simulink model "experiment_supervisor"  (R2025b)
settings: Solver=FixedStepDiscrete  StartTime=0.0  StopTime=inf  FixedStep=Ts  RelTol=1e-3
model workspace (MAT data in the model file):
  Ts = Simulink.Parameter
  Ts.Value = 0.01
  Ts.Complexity = 'real'
  Ts.Dimensions = [1 1]
  Ts.DataType = 'auto'
  Ts.DocUnits = 's'
  board_ID = Simulink.Parameter
  board_ID.Value = 1
  board_ID.Complexity = 'real'
  board_ID.Dimensions = [1 1]
  board_ID.DataType = 'auto'
undefined symbols (not defined in the file or in its folder): CAN_ANGLE_DEG2ICUB, CAN_ANGLE_ICUB2DEG, canChannel
libraries: canmsglib x21, canlib x4, simulink x1
settings Model: DataDictionary=amcbldc.sldd  Creator=upattacini  LastModifiedBy=rpumpo
settings SolverCC: AlgebraicLoopSolver=TrustRegion  DecoupledContinuousIntegration=on  MinimalZcImpactIntegration=on
settings OptimizationCC: ReuseModelBlockBuffer=off  SimCompilerOptimization=on
settings DebuggingCC: ParameterPrecisionLossMsg=none  UnconnectedInputMsg=warning  UnconnectedOutputMsg=warning  UnconnectedLineMsg=warning  ArithmeticOperatorsInVariantConditions=warning
settings HardwareCC: ProdBitPerLong=64.0  ProdHWDeviceType=Intel->x86-64 (Linux 64)
settings ModelReferenceCC: EnableRefExpFcnMdlSchedulingChecks=on
settings SFSimCC: SimUseLocalCustomCode=off  CustomCodeUndefinedFunction=UseInterfaceOnly
settings RTWCC: SystemTargetFile=sldrt.tlc  TemplateMakefile=sldrt.tmf  RTWUseLocalCustomCode=off  RTWCompilerOptimization=on  GPUComputeCapability=3.5  DLArmComputeVersion=19.05  Description=Simulink Desktop Real-Time
settings CodeAppCC: MaxIdLength=95.0
settings SimulinkDesktopRealTimeCC: ExtModeTransport=0.0  ExtModeStaticAllocSize=1000000.0  TargetLibSuffix=_sldrt.a  TargetPreCompLibLocation=C:\Program Files\MATLAB\R2025b\toolbox\sldrt\lib\win64  MultiwordLength=2048.0  DynamicStringBufferSize=256.0  ParMdlRefBuildCompliant=on  PreserveMATLABNamespacesInGeneratedCode=on  SubcomponentCodeInterfacePackaging=Reusable function

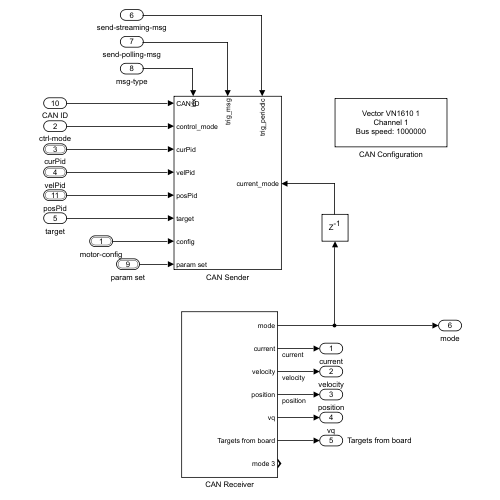
[thumbnail: Simulink's stored preview of the top-level diagram]
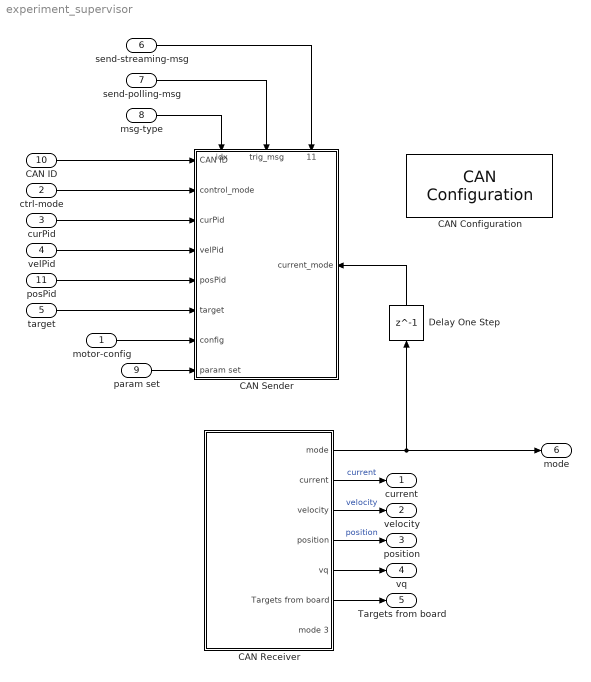
== system experiment_supervisor ==
  motor-config : Inport  OutDataTypeStr=Bus: MotorConfigurationExternal
  ctrl-mode : Inport  Port=2  OutDataTypeStr=Enum: MCControlModes
  curPid : Inport  Port=3  OutDataTypeStr=Bus: PID
  velPid : Inport  Port=4  OutDataTypeStr=Bus: PID
  target : Inport  Port=5
  send-streaming-msg : Inport  Port=6  OutDataTypeStr=uint8
  send-polling-msg : Inport  Port=7  OutDataTypeStr=uint8
  msg-type : Inport  Port=8  OutDataTypeStr=uint8
  param set : Inport  Port=9  OutDataTypeStr=Bus: MotorConfigurationExtSet
  CAN ID : Inport  Port=10
  posPid : Inport  Port=11  OutDataTypeStr=Bus: PID
  CAN Configuration : canlib/CAN Configuration  BlockHandle=6361.001  Device=Vector VN1610 1 (Channel 1)  DeviceMenu=Vector VN1610 1 (Channel 1)  ObjConstructor=canChannel('Vector', 'VN1610 1', 1)  BusSpeed=1000000  EnableBitParameters=off  SJW=1  TSEG1=4  TSEG2=3  NSamples=1  AckMode=Normal
  CAN Receiver : Subsystem
  CAN Sender : Subsystem
      settings: PortSchema="{\"entries\":[{\"content\":{\"sides\":[{\"content\":{\"connectorIds\":[\"In1\",\"In2\",\"In3\",\"In4\",\"In5\",\"In6\",\"In7\",\"In8\"]},\"type\":\"ConnectorPlacement.EquallySpacedRectSide\",\"uuid\":\"bdd6ce9e-9b65-4aba-9b48-f09f8c1326bb\"},{\"content\":{\"connectorIds\":[\"In12\"],\"side\":\"RIGHT\"},\"type\":\"ConnectorPlacement.EquallySpacedRectSide\",\"uuid\":\"141c9ef5-f742-47fc-b635-015c7474b58f\"},{\"content\":{\"connectorIds\":[\"In9\",\"In10\",\"In11\"],\"side\":\"TOP\"},\"type\":\"ConnectorPlacement.EquallySpacedRectSide\",\"uuid\":\"624889ac-74c5-4b05-9d21-0587daea952f\"}]},\"type\":\"ConnectorPlacement.EquallySpacedConnector\",\"uuid\":\"a748afda-e52d-41b4-a312-ee668058905d\"}],\"packageUris\":[\"http://schema.mathworks.com/mf0/Connector/R2020b\"],\"version\":\"1.0\"}"
  Delay One Step : Delay  DelayLength=1
  current : Outport
  velocity : Outport  Port=2
  position : Outport  Port=3
  vq : Outport  Port=4
  Targets from board : Outport  Port=5
  mode : Outport  Port=6
  wires:
  CAN Receiver/2(current) -> current/1  "current"
  CAN Receiver/3(velocity) -> velocity/1  "velocity"
  CAN Receiver/4(position) -> position/1  "position"
  CAN Receiver/5(vq) -> vq/1
  ctrl-mode/1 -> CAN Sender/2(control_mode)
  send-streaming-msg/1 -> CAN Sender/11(trig_periodic)
  CAN Receiver/6(Targets from board) -> Targets from board/1
  velPid/1 -> CAN Sender/4(velPid)
  curPid/1 -> CAN Sender/3(curPid)
  motor-config/1 -> CAN Sender/7(config)
  Delay One Step/1 -> CAN Sender/12(current_mode)
  send-polling-msg/1 -> CAN Sender/10(trig_msg)
  msg-type/1 -> CAN Sender/9(idx)
  target/1 -> CAN Sender/6(target)
  CAN ID/1 -> CAN Sender/1(CAN ID)
  CAN Receiver/1(mode) -> Delay One Step/1, mode/1
  param set/1 -> CAN Sender/8(param set)
  posPid/1 -> CAN Sender/5(posPid)

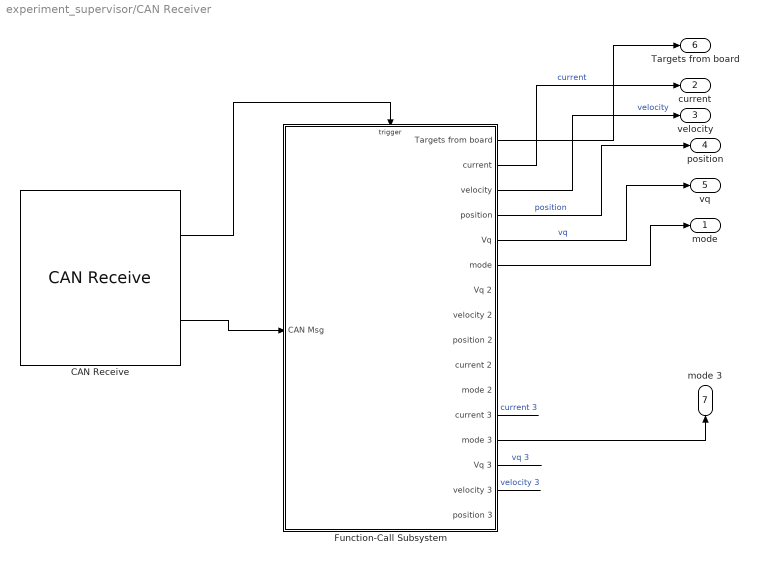
== system experiment_supervisor/CAN Receiver ==
  CAN Receive : canlib/CAN Receive  BlockHandle=6370.0007  Device=Vector VN1610 1 (Channel 1)  DeviceMenu=Vector VN1610 1 (Channel 1)  ObjConstructor=canChannel('Vector', 'VN1610 1', 1)  EnableStandardIDsFilter=off  StdIDsCombo=Allow all  StandardIDs=0  EnableExtendedIDsFilter=off  ExtIDsCombo=Allow all  ExtendedIDs=0  SampleTime=Ts  MsgsPerTimestep=all  InternalFilterUpdateStatus=on  BusOutput=on
  Function-Call Subsystem : Subsystem  TreatAsAtomicUnit=on
  mode : Outport
  current : Outport  Port=2
  velocity : Outport  Port=3
  position : Outport  Port=4
  vq : Outport  Port=5
  Targets from board : Outport  Port=6
  mode 3 : Outport  Port=7
  wires:
  CAN Receive/1 -> Function-Call Subsystem/Trigger
  CAN Receive/2 -> Function-Call Subsystem/1(CAN Msg)
  Function-Call Subsystem/2(current) -> current/1  "current"
  Function-Call Subsystem/3(velocity) -> velocity/1  "velocity"
  Function-Call Subsystem/4(position) -> position/1  "position"
  Function-Call Subsystem/5(Vq) -> vq/1  "vq"
  Function-Call Subsystem/1(Targets from board) -> Targets from board/1
  Function-Call Subsystem/6(mode) -> mode/1
  Function-Call Subsystem/12(current 3) -> ?  "current 3"
  Function-Call Subsystem/14(Vq 3) -> ?  "vq 3"
  Function-Call Subsystem/15(velocity 3) -> ?  "velocity 3"
  Function-Call Subsystem/13(mode 3) -> mode 3/1

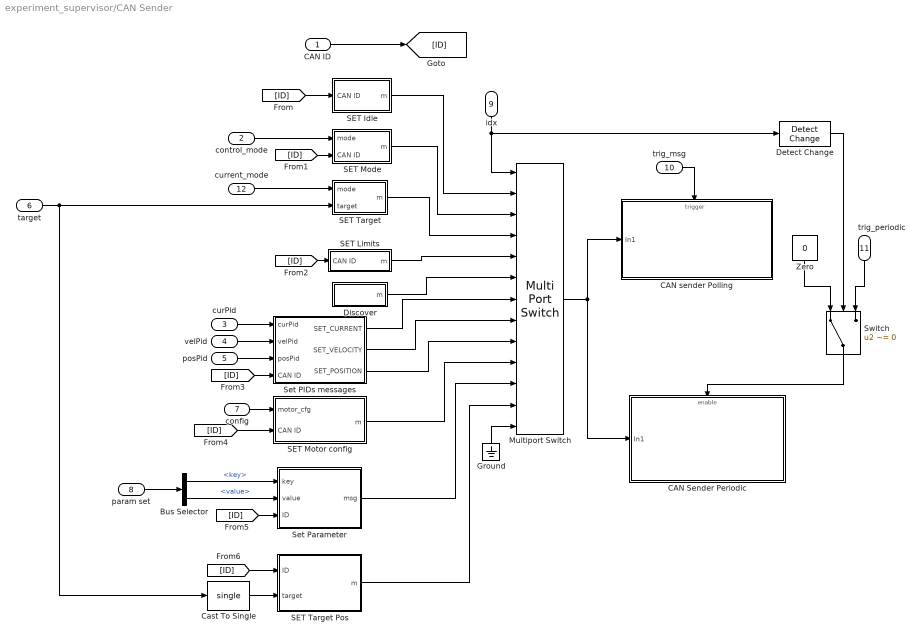
== system experiment_supervisor/CAN Sender ==
  CAN ID : Inport
  control_mode : Inport  Port=2
  curPid : Inport  Port=3
  velPid : Inport  Port=4
  posPid : Inport  Port=5
  target : Inport  Port=6
  config : Inport  Port=7
  param set : Inport  Port=8  OutDataTypeStr=Bus: MotorConfigurationExtSet
  idx : Inport  Port=9
  trig_msg : Inport  Port=10
  trig_periodic : Inport  Port=11
  current_mode : Inport  Port=12
  Bus Selector : BusSelector  OutputSignals=key,value
  CAN Sender Periodic : Subsystem  TreatAsAtomicUnit=on
  CAN sender Polling : Subsystem
  Cast To Single : DataTypeConversion  OutDataTypeStr=single  SaturateOnIntegerOverflow=off  RndMeth=Floor
  Detect Change : simulink/Logic and Bit Operations/Detect Change  vinit=0  OutDataTypeStr=boolean
  Discover : Subsystem
  Ground : Ground
  Multiport Switch : MultiPortSwitch  Inputs=11  DataPortForDefault=Additional data port  DiagnosticForDefault=None  SaturateOnIntegerOverflow=off  InputSameDT=off
  SET Idle : Subsystem
  SET Limits : Subsystem
  SET Mode : Subsystem
  SET Motor config : Subsystem
  SET Target : Subsystem
  SET Target Pos : Subsystem
  Set PIDs messages : Subsystem
  Set Parameter : Subsystem
  Switch : Switch  Criteria=u2 ~= 0  SaturateOnIntegerOverflow=off  InputSameDT=off
  Zero : Constant  Value=0  OutDataTypeStr=Inherit: Inherit via back propagation
  wires:
  idx/1 -> Multiport Switch/1, Detect Change/1
  trig_msg/1 -> CAN sender Polling/Trigger
  trig_periodic/1 -> Switch/3
  Multiport Switch/1 -> CAN sender Polling/1(In1), CAN Sender Periodic/1(In1)
  Set PIDs messages/2(SET_VELOCITY) -> Multiport Switch/8
  Set PIDs messages/1(SET_CURRENT) -> Multiport Switch/7
  velPid/1 -> Set PIDs messages/2(velPid)
  curPid/1 -> Set PIDs messages/1(curPid)
  Detect Change/1 -> Switch/2
  Zero/1 -> Switch/1
  Switch/1 -> CAN Sender Periodic/Enable
  SET Limits/1(m) -> Multiport Switch/5
  current_mode/1 -> SET Target/1(mode)
  target/1 -> Cast To Single/1, SET Target/2(target)
  SET Target/1(m) -> Multiport Switch/4
  config/1 -> SET Motor config/1(motor_cfg)
  SET Motor config/1(m) -> Multiport Switch/10
  control_mode/1 -> SET Mode/1(mode)
  SET Mode/1(m) -> Multiport Switch/3
  SET Idle/1(m) -> Multiport Switch/2
  Discover/1(m) -> Multiport Switch/6
  [ID] -> SET Idle/1(CAN ID)
  [ID] -> SET Mode/2(CAN ID)
  [ID] -> SET Limits/1(CAN ID)
  [ID] -> Set PIDs messages/4(CAN ID)
  [ID] -> SET Motor config/2(CAN ID)
  CAN ID/1 -> [ID]
  Set Parameter/1(msg) -> Multiport Switch/11
  [ID] -> Set Parameter/3(ID)
  param set/1 -> Bus Selector/1
  Bus Selector/1 -> Set Parameter/1(key)  "<key>"
  Bus Selector/2 -> Set Parameter/2(value)  "<value>"
  posPid/1 -> Set PIDs messages/3(posPid)
  Ground/1 -> Multiport Switch/13
  Set PIDs messages/3(SET_POSITION) -> Multiport Switch/9
  Cast To Single/1 -> SET Target Pos/2(target)
  [ID] -> SET Target Pos/1(ID)
  SET Target Pos/1(m) -> Multiport Switch/12

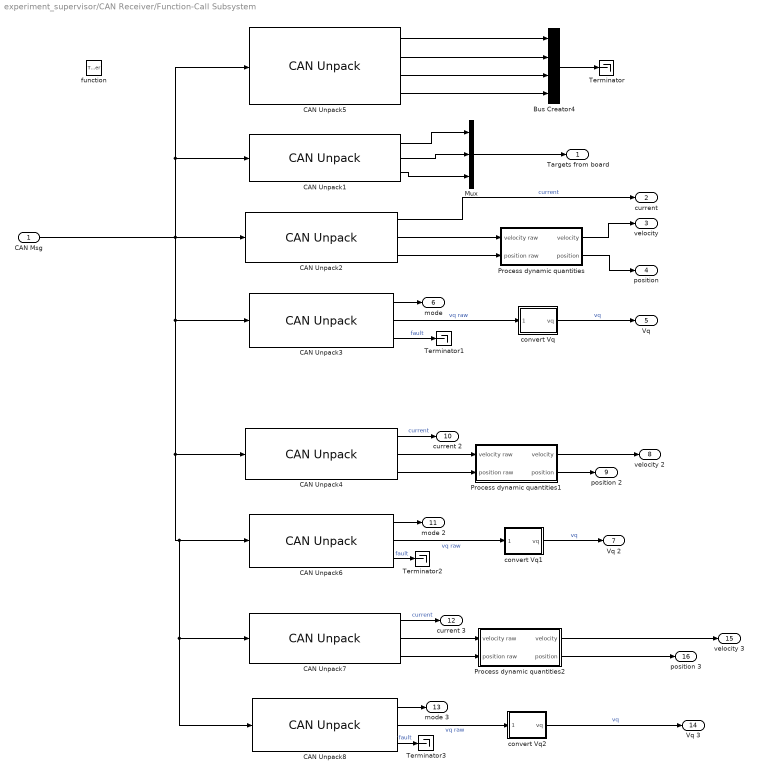
== system experiment_supervisor/CAN Receiver/Function-Call Subsystem ==
  CAN Msg : Inport
  function : TriggerPort  TriggerType=function-call  VariantControl=(inherit)
  Bus Creator4 : BusCreator  Inputs=4
  CAN Unpack1 : canmsglib/CAN Unpack  MsgList=(none)  MsgName=TARGETS  MsgIDType=Standard (11-bit identifier)  MsgIdentifier=0x10F  MsgLength=8  SignalInfo={ 'Target1', '0', '16', 'LE', 'signed', 'Standard', '0', '1', '0', '-Inf', 'Inf'; 'Target2', '16', '16', 'LE', 'signed', 'Standard', '0', '1', '0', '-Inf', 'Inf'; 'Target3', '32', '16', 'LE', 'signed', 'Standard', '0', '1', '0', '-Inf', 'Inf' }  IDPort=off  TimestampPort=off  ErrorPort=off  RemotePort=off  LengthPort=off  StatusPort=off  ApplyMinMax=off
  CAN Unpack2 : canmsglib/CAN Unpack  MsgList=(none)  MsgName=FOC  MsgIDType=Standard (11-bit identifier)  MsgIdentifier=0x110  MsgLength=8  SignalInfo={ 'current', '0', '16', 'LE', 'signed', 'Standard', '0', '1', '0', '-Inf', 'Inf'; 'velocity', '16', '16', 'LE', 'signed', 'Standard', '0', '1', '0', '-Inf', 'Inf'; 'position', '32', '32', 'LE', 'signed', 'Standard', '0', '1', '0', '-Inf', 'Inf' }  IDPort=off  TimestampPort=off  ErrorPort=off  RemotePort=off  LengthPort=off  StatusPort=off  ApplyMinMax=off
  CAN Unpack3 : canmsglib/CAN Unpack  MsgList=(none)  MsgName=STATUS  MsgIDType=Standard (11-bit identifier)  MsgIdentifier=0x113  MsgLength=8  SignalInfo={ 'mode', '0', '8', 'LE', 'unsigned', 'Standard', '0', '1', '0', '-Inf', 'Inf'; 'pwm', '16', '16', 'LE', 'unsigned', 'Standard', '0', '1', '0', '-Inf', 'Inf'; 'fault', '32', '8', 'LE', 'unsigned', 'Standard', '0', '1', '0', '-Inf', 'Inf' }  IDPort=off  TimestampPort=off  ErrorPort=off  RemotePort=off  LengthPort=off  StatusPort=off  ApplyMinMax=off
  CAN Unpack4 : canmsglib/CAN Unpack  MsgList=(none)  MsgName=FOC  MsgIDType=Standard (11-bit identifier)  MsgIdentifier=0x120  MsgLength=8  SignalInfo={ 'current', '0', '16', 'LE', 'signed', 'Standard', '0', '1', '0', '-Inf', 'Inf'; 'velocity', '16', '16', 'LE', 'signed', 'Standard', '0', '1', '0', '-Inf', 'Inf'; 'position', '32', '32', 'LE', 'signed', 'Standard', '0', '1', '0', '-Inf', 'Inf' }  IDPort=off  TimestampPort=off  ErrorPort=off  RemotePort=off  LengthPort=off  StatusPort=off  ApplyMinMax=off
  CAN Unpack5 : canmsglib/CAN Unpack  MsgList=(none)  MsgName=DISCOVER  MsgIDType=Standard (11-bit identifier)  MsgIdentifier=0x710  MsgLength=5  SignalInfo={}  IDPort=on  TimestampPort=on  ErrorPort=off  RemotePort=off  LengthPort=on  StatusPort=off  ApplyMinMax=off
      settings: DataFormat=raw data
  CAN Unpack6 : canmsglib/CAN Unpack  MsgList=(none)  MsgName=STATUS  MsgIDType=Standard (11-bit identifier)  MsgIdentifier=0x123  MsgLength=8  SignalInfo={ 'mode', '0', '8', 'LE', 'unsigned', 'Standard', '0', '1', '0', '-Inf', 'Inf'; 'pwm', '16', '16', 'LE', 'unsigned', 'Standard', '0', '1', '0', '-Inf', 'Inf'; 'fault', '32', '8', 'LE', 'unsigned', 'Standard', '0', '1', '0', '-Inf', 'Inf' }  IDPort=off  TimestampPort=off  ErrorPort=off  RemotePort=off  LengthPort=off  StatusPort=off  ApplyMinMax=off
  CAN Unpack7 : canmsglib/CAN Unpack  MsgList=(none)  MsgName=FOC  MsgIDType=Standard (11-bit identifier)  MsgIdentifier=0x130  MsgLength=8  SignalInfo={ 'current', '0', '16', 'LE', 'signed', 'Standard', '0', '1', '0', '-Inf', 'Inf'; 'velocity', '16', '16', 'LE', 'signed', 'Standard', '0', '1', '0', '-Inf', 'Inf'; 'position', '32', '32', 'LE', 'signed', 'Standard', '0', '1', '0', '-Inf', 'Inf' }  IDPort=off  TimestampPort=off  ErrorPort=off  RemotePort=off  LengthPort=off  StatusPort=off  ApplyMinMax=off
  CAN Unpack8 : canmsglib/CAN Unpack  MsgList=(none)  MsgName=STATUS  MsgIDType=Standard (11-bit identifier)  MsgIdentifier=0x133  MsgLength=8  SignalInfo={ 'mode', '0', '8', 'LE', 'unsigned', 'Standard', '0', '1', '0', '-Inf', 'Inf'; 'pwm', '16', '16', 'LE', 'unsigned', 'Standard', '0', '1', '0', '-Inf', 'Inf'; 'fault', '32', '8', 'LE', 'unsigned', 'Standard', '0', '1', '0', '-Inf', 'Inf' }  IDPort=off  TimestampPort=off  ErrorPort=off  RemotePort=off  LengthPort=off  StatusPort=off  ApplyMinMax=off
  Mux : Mux  Inputs=3
  Process dynamic quantities : Subsystem
  Process dynamic quantities1 : Subsystem
  Process dynamic quantities2 : Subsystem
  Terminator{,1..3} (4 alike) : Terminator
  convert Vq : Subsystem
  convert Vq1 : Subsystem
  convert Vq2 : Subsystem
  Targets from board : Outport
  current : Outport  Port=2  Unit=mA
  velocity : Outport  Port=3  Unit=deg/s
  position : Outport  Port=4  Unit=deg
  Vq : Outport  Port=5  Unit=%  PortDimensions=1
  mode : Outport  Port=6  OutDataTypeStr=uint8
  Vq 2 : Outport  Port=7
  velocity 2 : Outport  Port=8
  position 2 : Outport  Port=9
  current 2 : Outport  Port=10  Unit=mA
  mode 2 : Outport  Port=11  OutDataTypeStr=uint8
  current 3 : Outport  Port=12  Unit=mA
  mode 3 : Outport  Port=13  OutDataTypeStr=uint8
  Vq 3 : Outport  Port=14
  velocity 3 : Outport  Port=15
  position 3 : Outport  Port=16
  wires:
  CAN Unpack5/4 -> Bus Creator4/4
  CAN Unpack5/3 -> Bus Creator4/3
  CAN Unpack5/2 -> Bus Creator4/2
  CAN Unpack5/1 -> Bus Creator4/1
  Bus Creator4/1 -> Terminator/1
  CAN Unpack1/1 -> Mux/1
  CAN Unpack1/2 -> Mux/2
  CAN Unpack1/3 -> Mux/3
  Mux/1 -> Targets from board/1
  CAN Unpack2/2 -> Process dynamic quantities/1(velocity raw)
  CAN Unpack2/1 -> current/1  "current"
  Process dynamic quantities/2(position) -> position/1
  Process dynamic quantities/1(velocity) -> velocity/1
  CAN Unpack2/3 -> Process dynamic quantities/2(position raw)
  CAN Unpack3/2 -> convert Vq/1(vq raw)  "vq raw"
  CAN Unpack3/1 -> mode/1
  convert Vq/1(vq) -> Vq/1  "vq"
  CAN Unpack3/3 -> Terminator1/1  "fault"
  CAN Unpack4/2 -> Process dynamic quantities1/1(velocity raw)
  CAN Unpack4/3 -> Process dynamic quantities1/2(position raw)
  CAN Unpack6/2 -> convert Vq1/1(vq raw)  "vq raw"
  Process dynamic quantities1/1(velocity) -> velocity 2/1
  Process dynamic quantities1/2(position) -> position 2/1
  convert Vq1/1(vq) -> Vq 2/1  "vq"
  CAN Unpack4/1 -> current 2/1  "current"
  CAN Unpack6/1 -> mode 2/1
  CAN Unpack6/3 -> Terminator2/1  "fault"
  CAN Unpack8/3 -> Terminator3/1  "fault"
  CAN Unpack8/2 -> convert Vq2/1(vq raw)  "vq raw"
  CAN Unpack7/3 -> Process dynamic quantities2/2(position raw)
  CAN Unpack7/1 -> current 3/1  "current"
  CAN Unpack8/1 -> mode 3/1
  CAN Unpack7/2 -> Process dynamic quantities2/1(velocity raw)
  CAN Msg/1 -> CAN Unpack5/1, CAN Unpack1/1, CAN Unpack8/1, CAN Unpack7/1, CAN Unpack6/1, CAN Unpack4/1, CAN Unpack3/1, CAN Unpack2/1
  Process dynamic quantities2/2(position) -> position 3/1
  Process dynamic quantities2/1(velocity) -> velocity 3/1
  convert Vq2/1(vq) -> Vq 3/1  "vq"

== system experiment_supervisor/CAN Sender/CAN Sender Periodic ==
  In1 : Inport
  Enable : EnablePort
  CAN Transmit : canlib/CAN Transmit  BlockHandle=6815.0006  Device=Vector VN1610 1 (Channel 1)  DeviceMenu=Vector VN1610 1 (Channel 1)  ObjConstructor=canChannel('Vector', 'VN1610 1', 1)  EnableEventTransmit=off  EnablePeriodicTransmit=on  MessagePeriod=Ts
  wires:
  In1/1 -> CAN Transmit/1

== system experiment_supervisor/CAN Sender/CAN sender Polling ==
  In1 : Inport
  Trigger : TriggerPort  VariantControl=(inherit)  PortDimensions=1
  CAN Transmit : canlib/CAN Transmit  BlockHandle=6832.001  Device=Vector VN1610 1 (Channel 1)  DeviceMenu=Vector VN1610 1 (Channel 1)  ObjConstructor=canChannel('Vector', 'VN1610 1', 1)  EnableEventTransmit=off  EnablePeriodicTransmit=off  MessagePeriod=1.000
  wires:
  In1/1 -> CAN Transmit/1

== system experiment_supervisor/CAN Sender/Discover ==
  CAN Pack4 : canmsglib/CAN Pack  MsgList=(none)  MsgName=DISCOVER  MsgIDType=Standard (11-bit identifier)  MsgIdentifier=0x70F  CANIDInput=off  MsgLength=1  Remote=off  ApplyMinMax=off  BusOutput=on  SignalInfo={}
      settings: DataFormat=raw data
  discover : Constant  Value=0xFF
  m : Outport
  wires:
  CAN Pack4/1 -> m/1
  discover/1 -> CAN Pack4/1

== system experiment_supervisor/CAN Sender/SET Idle ==
  CAN ID : Inport
  CAN Pack : canmsglib/CAN Pack  MsgList=(none)  MsgName=CAN Idle  MsgIDType=Standard (11-bit identifier)  MsgIdentifier=board_ID  CANIDInput=on  MsgLength=2  Remote=off  ApplyMinMax=off  BusOutput=on  SignalInfo={ 'Idle', '0', '16', 'LE', 'unsigned', 'Standard', '0', '1', '0', '-Inf', 'Inf' }
      settings: DataFormat=manually specified signals
  idle-mode : Constant  Value=0x09  OutDataTypeStr=Inherit: Inherit via back propagation
  m : Outport
  wires:
  idle-mode/1 -> CAN Pack/1
  CAN ID/1 -> CAN Pack/2
  CAN Pack/1 -> m/1

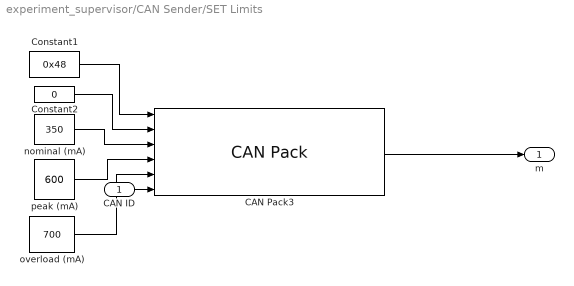
== system experiment_supervisor/CAN Sender/SET Limits ==
  CAN ID : Inport
  CAN Pack3 : canmsglib/CAN Pack  MsgList=(none)  MsgName=CAN Limits  MsgIDType=Standard (11-bit identifier)  MsgIdentifier=board_ID  CANIDInput=on  MsgLength=8  Remote=off  ApplyMinMax=off  BusOutput=on  SignalInfo={ 'CMD', '0', '8', 'LE', 'unsigned', 'Standard', '0', '1', '0', '-Inf', 'Inf'; 'X', '8', '8', 'LE', 'unsigned', 'Standard', '0', '1', '0', '-Inf', 'Inf'; 'NOMINAL', '16', '16', 'LE', 'unsigned', 'Standard', '0', '1', '0', '-Inf', 'Inf'; 'PEAK', '32', '16', 'LE', 'unsigned', 'Standard', '0', '1', '0', '-Inf', 'Inf'; 'OVERLOAD', '48', '16', 'LE', 'unsigned', 'Standard', '0', '1', '0', '-Inf', 'Inf' }
      settings: DataFormat=manually specified signals
  Constant1 : Constant  Value=0x48  OutDataTypeStr=Inherit: Inherit via back propagation
  Constant2 : Constant  Value=0  OutDataTypeStr=Inherit: Inherit via back propagation
  nominal (mA) : Constant  Value=350  OutDataTypeStr=Inherit: Inherit via back propagation
  overload (mA) : Constant  Value=700  OutDataTypeStr=Inherit: Inherit via back propagation
  peak (mA) : Constant  Value=600  OutDataTypeStr=Inherit: Inherit via back propagation
  m : Outport
  wires:
  Constant2/1 -> CAN Pack3/2
  Constant1/1 -> CAN Pack3/1
  nominal (mA)/1 -> CAN Pack3/3
  overload (mA)/1 -> CAN Pack3/5
  peak (mA)/1 -> CAN Pack3/4
  CAN ID/1 -> CAN Pack3/6
  CAN Pack3/1 -> m/1

== system experiment_supervisor/CAN Sender/SET Mode ==
  mode : Inport
  CAN ID : Inport  Port=2
  CAN Pack1 : canmsglib/CAN Pack  MsgList=(none)  MsgName=SET Control Mode  MsgIDType=Standard (11-bit identifier)  MsgIdentifier=board_ID  CANIDInput=on  MsgLength=2  Remote=off  ApplyMinMax=off  BusOutput=on  SignalInfo={ 'CMD', '0', '8', 'LE', 'unsigned', 'Standard', '0', '1', '0', '-Inf', 'Inf'; 'CTRL', '8', '8', 'LE', 'signed', 'Standard', '0', '1', '0', '-Inf', 'Inf' }
      settings: DataFormat=manually specified signals
  Cast : DataTypeConversion  OutDataTypeStr=uint8  SaturateOnIntegerOverflow=off  RndMeth=Floor
  current-mode : Constant  Value=0x09  OutDataTypeStr=Inherit: Inherit via back propagation
  m : Outport
  wires:
  current-mode/1 -> CAN Pack1/1
  Cast/1 -> CAN Pack1/2
  mode/1 -> Cast/1
  CAN ID/1 -> CAN Pack1/3
  CAN Pack1/1 -> m/1

== system experiment_supervisor/CAN Sender/SET Motor config ==
  motor_cfg : Inport
  CAN ID : Inport  Port=2
  CAN Pack5 : canmsglib/CAN Pack  MsgList=(none)  MsgName=Set_Motor_Config  MsgIDType=Standard (11-bit identifier)  MsgIdentifier=board_ID  CANIDInput=on  MsgLength=8  Remote=off  ApplyMinMax=off  BusOutput=on  SignalInfo={ 'CMD', '0', '8', 'LE', 'unsigned', 'Standard', '0', '1', '0', '-Inf', 'Inf'; 'FLAGS', '8', '8', 'LE', 'unsigned', 'Standard', '0', '1', '0', '-Inf', 'Inf'; 'RES_ENCODER', '16', '16', 'LE', 'signed', 'Standard', '0', '1', '0', '-Inf', 'Inf'; 'OFFSET_ENCODER', '32', '16', 'LE', 'unsigned', 'Standard', '0', '1', '0', '-Inf', 'Inf'; 'N_POLES', '48', '8', 'LE', 'unsigned', 'Standard', '0', '1', '0', '-Inf', 'Inf'; 'ENCODER_TOLERANCE', '56', '8', 'LE', 'unsigned', 'Standard', '0', '1', '0', '-Inf', 'Inf' }
      settings: DataFormat=manually specified signals
  Constant3 : Constant  Value=0x77  OutDataTypeStr=Inherit: Inherit via back propagation
  Unpack motor configuration : MATLAB Function  TreatAsAtomicUnit=on
  m : Outport
  wires:
  motor_cfg/1 -> Unpack motor configuration/1(motor_cfg)
  Unpack motor configuration/2(resolution) -> CAN Pack5/3
  Unpack motor configuration/3(rotor_offset) -> CAN Pack5/4
  Unpack motor configuration/1(flags) -> CAN Pack5/2
  Unpack motor configuration/4(n_poles) -> CAN Pack5/5
  Unpack motor configuration/5(enc_tolerance) -> CAN Pack5/6
  Constant3/1 -> CAN Pack5/1
  CAN ID/1 -> CAN Pack5/7
  CAN Pack5/1 -> m/1

== system experiment_supervisor/CAN Sender/SET Target ==
  mode : Inport
  target : Inport  Port=2
  CAN Pack2 : canmsglib/CAN Pack  MsgList=(none)  MsgName=CAN Target  MsgIDType=Standard (11-bit identifier)  MsgIdentifier=0x10F  CANIDInput=off  MsgLength=8  Remote=off  ApplyMinMax=off  BusOutput=on  SignalInfo={ 'Target 1', '0', '16', 'LE', 'signed', 'Standard', '0', '1', '0', '-Inf', 'Inf'; 'Target 2', '16', '16', 'LE', 'signed', 'Standard', '0', '1', '0', '-Inf', 'Inf'; 'Target 3', '32', '16', 'LE', 'signed', 'Standard', '0', '1', '0', '-Inf', 'Inf'; 'Target 4', '48', '16', 'LE', 'signed', 'Standard', '0', '1', '0', '-Inf', 'Inf' }
      settings: DataFormat=manually specified signals
  Cast To Single : DataTypeConversion  OutDataTypeStr=single  SaturateOnIntegerOverflow=off  RndMeth=Floor
  Cast1 : DataTypeConversion  OutDataTypeStr=Enum: MCControlModes  SaturateOnIntegerOverflow=off  RndMeth=Floor
  Target conditioning : Subsystem
  m : Outport
  wires:
  Target conditioning/1(out) -> CAN Pack2/1, CAN Pack2/2, CAN Pack2/4, CAN Pack2/3  "target"
  Cast To Single/1 -> Target conditioning/2(tg)
  Cast1/1 -> Target conditioning/1(control_mode)
  target/1 -> Cast To Single/1
  CAN Pack2/1 -> m/1
  mode/1 -> Cast1/1

== system experiment_supervisor/CAN Sender/SET Target Pos ==
  ID : Inport
  target : Inport  Port=2
  CAN Pack2 : canmsglib/CAN Pack  MsgList=(none)  MsgName=SET  MsgIDType=Standard (11-bit identifier)  MsgIdentifier=0x10F  CANIDInput=on  MsgLength=8  Remote=off  ApplyMinMax=off  BusOutput=on  SignalInfo={ 'CMD', '0', '8', 'LE', 'unsigned', 'Standard', '0', '1', '0', '-Inf', 'Inf'; 'SetPos', '8', '8', 'LE', 'unsigned', 'Standard', '0', '1', '0', '-Inf', 'Inf'; 'TargetPos', '16', '32', 'LE', 'single', 'Standard', '0', '1', '0', '-Inf', 'Inf'; 'Vel', '48', '16', 'LE', 'unsigned', 'Standard', '0', '1', '0', '-Inf', 'Inf' }
      settings: DataFormat=manually specified signals
  Constant : Constant  Value=0x70e2  OutDataTypeStr=uint16
  Constant1 : Constant  Value=0x05
  Target conditioning : Subsystem
  m : Outport
  wires:
  target/1 -> Target conditioning/1(tg)
  CAN Pack2/1 -> m/1
  ID/1 -> CAN Pack2/5
  Constant/1 -> CAN Pack2/4
  Constant1/1 -> CAN Pack2/1
  Target conditioning/1(ID) -> CAN Pack2/2
  Target conditioning/2(Position) -> CAN Pack2/3

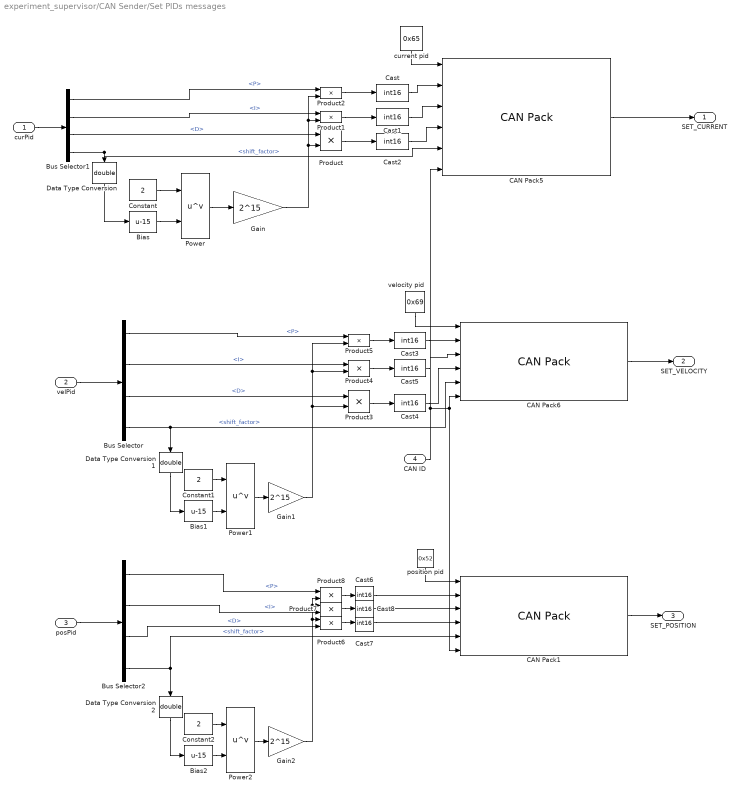
== system experiment_supervisor/CAN Sender/Set PIDs messages ==
  curPid : Inport
  velPid : Inport  Port=2
  posPid : Inport  Port=3
  CAN ID : Inport  Port=4
  Bias : Bias  Bias=-15  SaturateOnIntegerOverflow=off
  Bias1 : Bias  Bias=-15  SaturateOnIntegerOverflow=off
  Bias2 : Bias  Bias=-15  SaturateOnIntegerOverflow=off
  Bus Selector : BusSelector  OutputSignals=P,I,D,shift_factor
  Bus Selector1 : BusSelector  OutputSignals=P,I,D,shift_factor
  Bus Selector2 : BusSelector  OutputSignals=P,I,D,shift_factor
  CAN Pack1 : canmsglib/CAN Pack  MsgList=(none)  MsgName=SET_VELOCITY_PID  MsgIDType=Standard (11-bit identifier)  MsgIdentifier=board_ID  CANIDInput=on  MsgLength=8  Remote=off  ApplyMinMax=off  BusOutput=on  SignalInfo={ 'CMD', '0', '8', 'LE', 'unsigned', 'Standard', '0', '1', '0', '-Inf', 'Inf'; 'Kp', '8', '16', 'LE', 'signed', 'Standard', '0', '1', '0', '-Inf', 'Inf'; 'Ki', '24', '16', 'LE', 'signed', 'Standard', '0', '1', '0', '-Inf', 'Inf'; 'Kd', '40', '16', 'LE', 'signed', 'Standard', '0', '1', '0', '-Inf', 'Inf'; 'shift', '56', '8', 'LE', 'unsigned', 'Standard', '0', '1', '0', '-Inf', 'Inf' }
      settings: DataFormat=manually specified signals
  CAN Pack5 : canmsglib/CAN Pack  MsgList=(none)  MsgName=SET_CURRENT_PID  MsgIDType=Standard (11-bit identifier)  MsgIdentifier=board_ID  CANIDInput=on  MsgLength=8  Remote=off  ApplyMinMax=off  BusOutput=on  SignalInfo={ 'CMD', '0', '8', 'LE', 'unsigned', 'Standard', '0', '1', '0', '-Inf', 'Inf'; 'Kp', '8', '16', 'LE', 'signed', 'Standard', '0', '1', '0', '-Inf', 'Inf'; 'Ki', '24', '16', 'LE', 'signed', 'Standard', '0', '1', '0', '-Inf', 'Inf'; 'Kd', '40', '16', 'LE', 'signed', 'Standard', '0', '1', '0', '-Inf', 'Inf'; 'shift', '56', '8', 'LE', 'unsigned', 'Standard', '0', '1', '0', '-Inf', 'Inf' }
      settings: DataFormat=manually specified signals
  CAN Pack6 : canmsglib/CAN Pack  MsgList=(none)  MsgName=SET_VELOCITY_PID  MsgIDType=Standard (11-bit identifier)  MsgIdentifier=board_ID  CANIDInput=on  MsgLength=8  Remote=off  ApplyMinMax=off  BusOutput=on  SignalInfo={ 'CMD', '0', '8', 'LE', 'unsigned', 'Standard', '0', '1', '0', '-Inf', 'Inf'; 'Kp', '8', '16', 'LE', 'signed', 'Standard', '0', '1', '0', '-Inf', 'Inf'; 'Ki', '24', '16', 'LE', 'signed', 'Standard', '0', '1', '0', '-Inf', 'Inf'; 'Kd', '40', '16', 'LE', 'signed', 'Standard', '0', '1', '0', '-Inf', 'Inf'; 'shift', '56', '8', 'LE', 'unsigned', 'Standard', '0', '1', '0', '-Inf', 'Inf' }
      settings: DataFormat=manually specified signals
  Cast{,1..8} (9 alike) : DataTypeConversion  OutDataTypeStr=int16  SaturateOnIntegerOverflow=off  RndMeth=Floor
  Constant : Constant  Value=2
  Constant1 : Constant  Value=2
  Constant2 : Constant  Value=2
  Data Type Conversion : DataTypeConversion  OutDataTypeStr=double  SaturateOnIntegerOverflow=off  RndMeth=Floor
  Data Type Conversion1 : DataTypeConversion  OutDataTypeStr=double  SaturateOnIntegerOverflow=off  RndMeth=Floor
  Data Type Conversion2 : DataTypeConversion  OutDataTypeStr=double  SaturateOnIntegerOverflow=off  RndMeth=Floor
  Gain : Gain  Gain=2^15  OutDataTypeStr=single
  Gain1 : Gain  Gain=2^15  OutDataTypeStr=single
  Gain2 : Gain  Gain=2^15  OutDataTypeStr=single
  Power : Math  Operator=pow
  Power1 : Math  Operator=pow
  Power2 : Math  Operator=pow
  Product{,1..8} (9 alike) : Product
  current pid : Constant  Value=0x65  OutDataTypeStr=int16
  position pid : Constant  Value=0x52  OutDataTypeStr=int16
  velocity pid : Constant  Value=0x69  OutDataTypeStr=int16
  SET_CURRENT : Outport
  SET_VELOCITY : Outport  Port=2
  SET_POSITION : Outport  Port=3
  wires:
  Bus Selector/4 -> CAN Pack6/5, Data Type Conversion1/1  "<shift_factor>"
  Bus Selector1/4 -> CAN Pack5/5, Data Type Conversion/1  "<shift_factor>"
  Bus Selector1/1 -> Product2/1  "<P>"
  Bus Selector1/2 -> Product1/1  "<I>"
  current pid/1 -> CAN Pack5/1
  velocity pid/1 -> CAN Pack6/1
  CAN Pack5/1 -> SET_CURRENT/1
  CAN Pack6/1 -> SET_VELOCITY/1
  velPid/1 -> Bus Selector/1
  curPid/1 -> Bus Selector1/1
  Bus Selector1/3 -> Product/1  "<D>"
  Power/1 -> Gain/1
  Gain/1 -> Product2/2, Product1/2, Product/2
  Product/1 -> Cast2/1
  Product1/1 -> Cast1/1
  Product2/1 -> Cast/1
  Cast/1 -> CAN Pack5/2
  Cast1/1 -> CAN Pack5/3
  Cast2/1 -> CAN Pack5/4
  Constant/1 -> Power/1
  Bias/1 -> Power/2
  Data Type Conversion/1 -> Bias/1
  Cast5/1 -> CAN Pack6/3
  Bus Selector/2 -> Product4/1  "<I>"
  Cast3/1 -> CAN Pack6/2
  Bus Selector/3 -> Product3/1  "<D>"
  Bus Selector/1 -> Product5/1  "<P>"
  Cast4/1 -> CAN Pack6/4
  CAN ID/1 -> CAN Pack6/6, CAN Pack1/6, CAN Pack5/6
  position pid/1 -> CAN Pack1/1
  posPid/1 -> Bus Selector2/1
  Gain1/1 -> Product3/2, Product5/2, Product4/2
  Bias1/1 -> Power1/2
  Data Type Conversion1/1 -> Bias1/1
  Constant1/1 -> Power1/1
  Power1/1 -> Gain1/1
  Product5/1 -> Cast3/1
  Product4/1 -> Cast5/1
  Product3/1 -> Cast4/1
  Constant2/1 -> Power2/1
  Bias2/1 -> Power2/2
  Data Type Conversion2/1 -> Bias2/1
  Gain2/1 -> Product8/2, Product7/1, Product6/1
  Power2/1 -> Gain2/1
  Bus Selector2/4 -> Data Type Conversion2/1, CAN Pack1/5  "<shift_factor>"
  Product6/1 -> Cast7/1
  Product8/1 -> Cast6/1
  Product7/1 -> Cast8/1
  Cast6/1 -> CAN Pack1/2
  Cast8/1 -> CAN Pack1/3
  Cast7/1 -> CAN Pack1/4
  Bus Selector2/3 -> Product6/2  "<D>"
  Bus Selector2/2 -> Product7/2  "<I>"
  Bus Selector2/1 -> Product8/1  "<P>"
  CAN Pack1/1 -> SET_POSITION/1

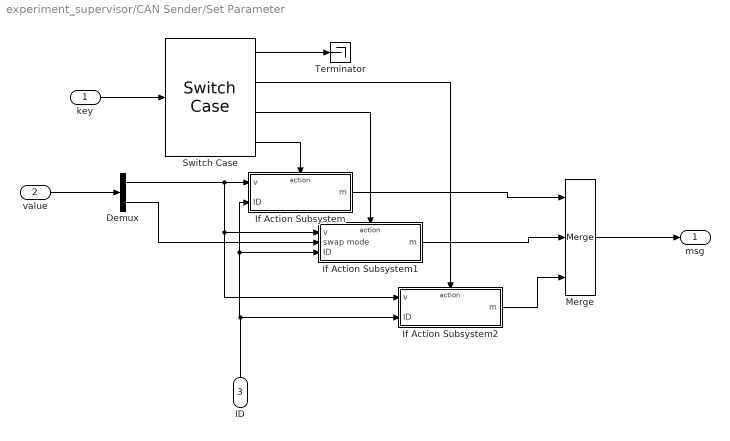
== system experiment_supervisor/CAN Sender/Set Parameter ==
  key : Inport
  value : Inport  Port=2
  ID : Inport  Port=3
  Demux : Demux  Outputs=2
  If Action Subsystem : Subsystem  TreatAsAtomicUnit=on
  If Action Subsystem1 : Subsystem  TreatAsAtomicUnit=on
  If Action Subsystem2 : Subsystem  TreatAsAtomicUnit=on
  Merge : Merge  Inputs=3
  Switch Case : SwitchCase  CaseConditions="{MCMotorParamsSet.None, MCMotorParamsSet.Kbemf, MCMotorParamsSet.hall,  MCMotorParamsSet.elect_vmax}"  ShowDefaultCase=off
  Terminator : Terminator
  msg : Outport
  wires:
  Merge/1 -> msg/1
  If Action Subsystem/1(m) -> Merge/1
  Demux/1 -> If Action Subsystem2/1(v), If Action Subsystem1/1(v), If Action Subsystem/1(v)
  key/1 -> Switch Case/1
  If Action Subsystem1/1(m) -> Merge/2
  If Action Subsystem2/1(m) -> Merge/3
  ID/1 -> If Action Subsystem/2(ID), If Action Subsystem1/3(ID), If Action Subsystem2/2(ID)
  Demux/2 -> If Action Subsystem1/2(swap mode)
  value/1 -> Demux/1
  Switch Case/2 -> If Action Subsystem2/Action
  Switch Case/3 -> If Action Subsystem1/Action
  Switch Case/4 -> If Action Subsystem/Action
  Switch Case/1 -> Terminator/1

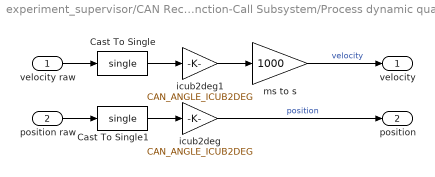
== system experiment_supervisor/CAN Receiver/Function-Call Subsystem/Process dynamic quantities ==
  velocity raw : Inport
  position raw : Inport  Port=2
  Cast To Single : DataTypeConversion  OutDataTypeStr=single  SaturateOnIntegerOverflow=off  RndMeth=Floor
  Cast To Single1 : DataTypeConversion  OutDataTypeStr=single  SaturateOnIntegerOverflow=off  RndMeth=Floor
  icub2deg : Gain  Gain=CAN_ANGLE_ICUB2DEG
  icub2deg1 : Gain  Gain=CAN_ANGLE_ICUB2DEG
  ms to s : Gain  Gain=1000
  velocity : Outport
  position : Outport  Port=2
  wires:
  Cast To Single1/1 -> icub2deg/1
  icub2deg1/1 -> ms to s/1
  Cast To Single/1 -> icub2deg1/1
  icub2deg/1 -> position/1  "position"
  velocity raw/1 -> Cast To Single/1
  position raw/1 -> Cast To Single1/1
  ms to s/1 -> velocity/1  "velocity"

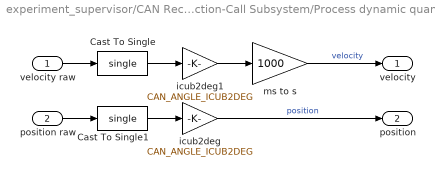
== system experiment_supervisor/CAN Receiver/Function-Call Subsystem/Process dynamic quantities1 ==
  velocity raw : Inport
  position raw : Inport  Port=2
  Cast To Single : DataTypeConversion  OutDataTypeStr=single  SaturateOnIntegerOverflow=off  RndMeth=Floor
  Cast To Single1 : DataTypeConversion  OutDataTypeStr=single  SaturateOnIntegerOverflow=off  RndMeth=Floor
  icub2deg : Gain  Gain=CAN_ANGLE_ICUB2DEG
  icub2deg1 : Gain  Gain=CAN_ANGLE_ICUB2DEG
  ms to s : Gain  Gain=1000
  velocity : Outport
  position : Outport  Port=2
  wires:
  Cast To Single1/1 -> icub2deg/1
  icub2deg1/1 -> ms to s/1
  Cast To Single/1 -> icub2deg1/1
  icub2deg/1 -> position/1  "position"
  velocity raw/1 -> Cast To Single/1
  position raw/1 -> Cast To Single1/1
  ms to s/1 -> velocity/1  "velocity"

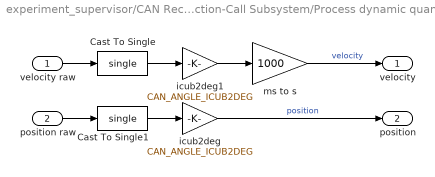
== system experiment_supervisor/CAN Receiver/Function-Call Subsystem/Process dynamic quantities2 ==
  velocity raw : Inport
  position raw : Inport  Port=2
  Cast To Single : DataTypeConversion  OutDataTypeStr=single  SaturateOnIntegerOverflow=off  RndMeth=Floor
  Cast To Single1 : DataTypeConversion  OutDataTypeStr=single  SaturateOnIntegerOverflow=off  RndMeth=Floor
  icub2deg : Gain  Gain=CAN_ANGLE_ICUB2DEG
  icub2deg1 : Gain  Gain=CAN_ANGLE_ICUB2DEG
  ms to s : Gain  Gain=1000
  velocity : Outport
  position : Outport  Port=2
  wires:
  Cast To Single1/1 -> icub2deg/1
  icub2deg1/1 -> ms to s/1
  Cast To Single/1 -> icub2deg1/1
  icub2deg/1 -> position/1  "position"
  velocity raw/1 -> Cast To Single/1
  position raw/1 -> Cast To Single1/1
  ms to s/1 -> velocity/1  "velocity"

== system experiment_supervisor/CAN Receiver/Function-Call Subsystem/convert Vq ==
  vq raw : Inport
  Data Type Conversion : DataTypeConversion  OutDataTypeStr=int16  SaturateOnIntegerOverflow=off  RndMeth=Floor
  Data Type Conversion1 : DataTypeConversion  OutDataTypeStr=single  SaturateOnIntegerOverflow=off  RndMeth=Floor
  Gain : Gain  Gain=1/32
  Gain1 : Gain  Gain=1/10
  vq : Outport
  wires:
  vq raw/1 -> Data Type Conversion/1
  Gain/1 -> Data Type Conversion1/1
  Data Type Conversion/1 -> Gain/1  "vq"
  Data Type Conversion1/1 -> Gain1/1
  Gain1/1 -> vq/1

== system experiment_supervisor/CAN Receiver/Function-Call Subsystem/convert Vq1 ==
  vq raw : Inport
  Data Type Conversion : DataTypeConversion  OutDataTypeStr=int16  SaturateOnIntegerOverflow=off  RndMeth=Floor
  Data Type Conversion1 : DataTypeConversion  OutDataTypeStr=single  SaturateOnIntegerOverflow=off  RndMeth=Floor
  Gain : Gain  Gain=1/32
  Gain1 : Gain  Gain=1/10
  vq : Outport
  wires:
  vq raw/1 -> Data Type Conversion/1
  Gain/1 -> Data Type Conversion1/1
  Data Type Conversion/1 -> Gain/1  "vq"
  Data Type Conversion1/1 -> Gain1/1
  Gain1/1 -> vq/1

== system experiment_supervisor/CAN Receiver/Function-Call Subsystem/convert Vq2 ==
  vq raw : Inport
  Data Type Conversion : DataTypeConversion  OutDataTypeStr=int16  SaturateOnIntegerOverflow=off  RndMeth=Floor
  Data Type Conversion1 : DataTypeConversion  OutDataTypeStr=single  SaturateOnIntegerOverflow=off  RndMeth=Floor
  Gain : Gain  Gain=1/32
  Gain1 : Gain  Gain=1/10
  vq : Outport
  wires:
  vq raw/1 -> Data Type Conversion/1
  Gain/1 -> Data Type Conversion1/1
  Data Type Conversion/1 -> Gain/1  "vq"
  Data Type Conversion1/1 -> Gain1/1
  Gain1/1 -> vq/1

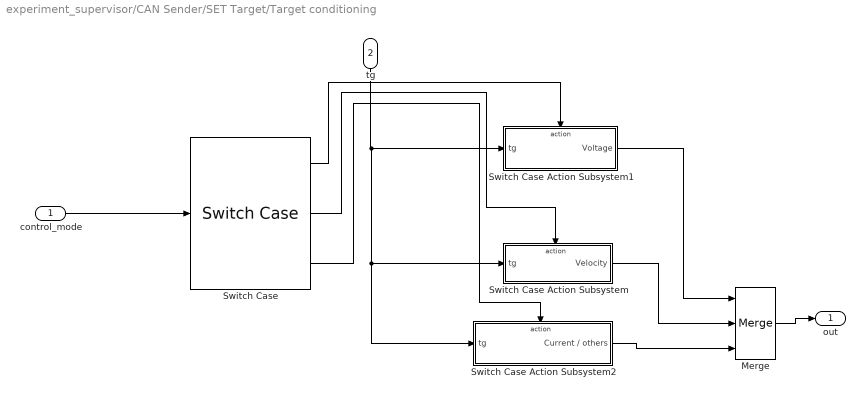
== system experiment_supervisor/CAN Sender/SET Target/Target conditioning ==
  control_mode : Inport
  tg : Inport  Port=2
  Merge : Merge  Inputs=3
  Switch Case : SwitchCase  CaseConditions={MCControlModes.OpenLoop, MCControlModes.SpeedVoltage}
  Switch Case Action Subsystem : Subsystem  TreatAsAtomicUnit=on
  Switch Case Action Subsystem1 : Subsystem  TreatAsAtomicUnit=on
  Switch Case Action Subsystem2 : Subsystem  TreatAsAtomicUnit=on
  out : Outport
  wires:
  tg/1 -> Switch Case Action Subsystem2/1(tg), Switch Case Action Subsystem/1(tg), Switch Case Action Subsystem1/1(tg)
  Switch Case/1 -> Switch Case Action Subsystem1/Action
  Switch Case/2 -> Switch Case Action Subsystem/Action
  Switch Case/3 -> Switch Case Action Subsystem2/Action
  Merge/1 -> out/1
  control_mode/1 -> Switch Case/1
  Switch Case Action Subsystem1/1(Voltage) -> Merge/1
  Switch Case Action Subsystem/1(Velocity) -> Merge/2
  Switch Case Action Subsystem2/1(Current / others) -> Merge/3

== system experiment_supervisor/CAN Sender/SET Target Pos/Target conditioning ==
  tg : Inport
  Zero : Constant  OutDataTypeStr=uint16
  ID : Outport
  Position : Outport  Port=2
  wires:
  tg/1 -> Position/1
  Zero/1 -> ID/1

== system experiment_supervisor/CAN Sender/Set Parameter/If Action Subsystem ==
  v : Inport
  ID : Inport  Port=2
  Action Port : ActionPort  ActionPortLabel=case [ elect_vmax ]:
  CAN Pack : canmsglib/CAN Pack  MsgList=(none)  MsgName=Set Value  MsgIDType=Standard (11-bit identifier)  MsgIdentifier=board_ID  CANIDInput=on  MsgLength=8  Remote=off  ApplyMinMax=off  BusOutput=on  SignalInfo={ 'OPC', '0', '8', 'LE', 'unsigned', 'Standard', '0', '1', '0', '-Inf', 'Inf'; 'value', '16', '32', 'LE', 'single', 'Standard', '0', '1', '0', '-Inf', 'Inf'; 'elec_vmax', '8', '8', 'LE', 'unsigned', 'Standard', '0', '1', '0', '-Inf', 'Inf' }
      settings: LibrarySourceBlock=stmutilitieslib/CAN Pack  DataFormat=manually specified signals
  Cast : DataTypeConversion  OutDataTypeStr=uint8  SaturateOnIntegerOverflow=off  RndMeth=Floor
  SET : Constant  Value=0x01  OutDataTypeStr=uint8
  elect_Vmax : Constant  Value=0x03  OutDataTypeStr=uint8
  m : Outport
  wires:
  v/1 -> Cast/1
  SET/1 -> CAN Pack/1
  ID/1 -> CAN Pack/4
  CAN Pack/1 -> m/1
  Cast/1 -> CAN Pack/2
  elect_Vmax/1 -> CAN Pack/3

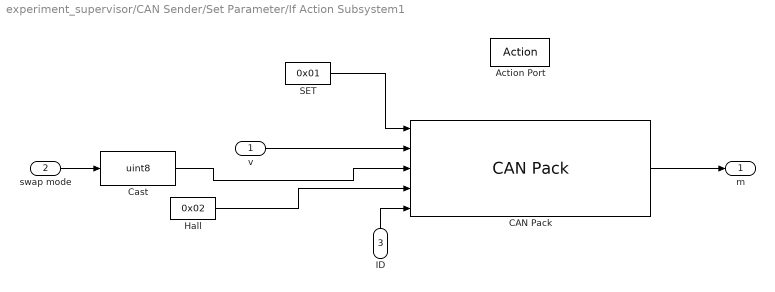
== system experiment_supervisor/CAN Sender/Set Parameter/If Action Subsystem1 ==
  v : Inport
  swap mode : Inport  Port=2
  ID : Inport  Port=3
  Action Port : ActionPort  ActionPortLabel=case [ hall ]:
  CAN Pack : canmsglib/CAN Pack  MsgList=(none)  MsgName=Set Value  MsgIDType=Standard (11-bit identifier)  MsgIdentifier=board_ID  CANIDInput=on  MsgLength=8  Remote=off  ApplyMinMax=off  BusOutput=on  SignalInfo={ 'OPC', '0', '8', 'LE', 'unsigned', 'Standard', '0', '1', '0', '-Inf', 'Inf'; 'offset', '16', '16', 'LE', 'unsigned', 'Standard', '0', '1', '0', '-Inf', 'Inf'; 'swap_mode', '32', '8', 'LE', 'unsigned', 'Standard', '0', '1', '0', '-Inf', 'Inf'; 'hall', '8', '8', 'LE', 'unsigned', 'Standard', '0', '1', '0', '-Inf', 'Inf' }
      settings: LibrarySourceBlock=stmutilitieslib/CAN Pack  DataFormat=manually specified signals
  Cast : DataTypeConversion  OutDataTypeStr=uint8  SaturateOnIntegerOverflow=off  RndMeth=Floor
  Hall : Constant  Value=0x02  OutDataTypeStr=uint8
  SET : Constant  Value=0x01  OutDataTypeStr=uint8
  m : Outport
  wires:
  CAN Pack/1 -> m/1
  SET/1 -> CAN Pack/1
  v/1 -> CAN Pack/2
  ID/1 -> CAN Pack/5
  swap mode/1 -> Cast/1
  Cast/1 -> CAN Pack/3
  Hall/1 -> CAN Pack/4

== system experiment_supervisor/CAN Sender/Set Parameter/If Action Subsystem2 ==
  v : Inport
  ID : Inport  Port=2
  Action Port : ActionPort  ActionPortLabel=case [ Kbemf ]:
  CAN Pack : canmsglib/CAN Pack  MsgList=(none)  MsgName=Set Value  MsgIDType=Standard (11-bit identifier)  MsgIdentifier=board_ID  CANIDInput=on  MsgLength=8  Remote=off  ApplyMinMax=off  BusOutput=on  SignalInfo={ 'OPC', '0', '8', 'LE', 'unsigned', 'Standard', '0', '1', '0', '-Inf', 'Inf'; 'value', '16', '32', 'LE', 'single', 'Standard', '0', '1', '0', '-Inf', 'Inf'; 'kbemf', '8', '8', 'LE', 'unsigned', 'Standard', '0', '1', '0', '-Inf', 'Inf' }
      settings: LibrarySourceBlock=stmutilitieslib/CAN Pack  DataFormat=manually specified signals
  Kbemf : Constant  Value=0x01  OutDataTypeStr=uint8
  SET : Constant  Value=0x01  OutDataTypeStr=uint8
  m : Outport
  wires:
  CAN Pack/1 -> m/1
  SET/1 -> CAN Pack/1
  v/1 -> CAN Pack/2
  ID/1 -> CAN Pack/4
  Kbemf/1 -> CAN Pack/3

== system experiment_supervisor/CAN Sender/SET Target/Target conditioning/Switch Case Action Subsystem ==
  tg : Inport
  Action Port : ActionPort  ActionPortLabel=case [ SpeedVoltage ]:
  Data Type Conversion2 : DataTypeConversion  OutDataTypeStr=int16  SaturateOnIntegerOverflow=off  RndMeth=Floor
  Gain : Gain  Gain=1/1000
  Product : Product
  deg2icub : Constant  Value=CAN_ANGLE_DEG2ICUB  OutDataTypeStr=single
  Velocity : Outport
  wires:
  tg/1 -> Product/2
  Gain/1 -> Product/1
  deg2icub/1 -> Gain/1
  Product/1 -> Data Type Conversion2/1
  Data Type Conversion2/1 -> Velocity/1

== system experiment_supervisor/CAN Sender/SET Target/Target conditioning/Switch Case Action Subsystem1 ==
  tg : Inport
  Action Port : ActionPort  ActionPortLabel=case [ OpenLoop ]:
  Data Type Conversion : DataTypeConversion  OutDataTypeStr=int16  SaturateOnIntegerOverflow=off  RndMeth=Floor
  Gain : Gain  Gain=32
  Gain1 : Gain  Gain=10
  Voltage : Outport
  wires:
  Gain1/1 -> Gain/1
  tg/1 -> Gain1/1
  Data Type Conversion/1 -> Voltage/1
  Gain/1 -> Data Type Conversion/1

== system experiment_supervisor/CAN Sender/SET Target/Target conditioning/Switch Case Action Subsystem2 ==
  tg : Inport
  Action Port : ActionPort  ActionPortLabel=default:
  Data Type Conversion3 : DataTypeConversion  OutDataTypeStr=int16  SaturateOnIntegerOverflow=off  RndMeth=Floor
  Current / others : Outport
  wires:
  tg/1 -> Data Type Conversion3/1
  Data Type Conversion3/1 -> Current / others/1

== matlab function experiment_supervisor/CAN Sender/SET Motor config/Unpack motor configuration ==
  data: flags output; resolution output; rotor_offset output; n_poles output; motor_cfg input; enc_tolerance output
function [flags, resolution,rotor_offset, n_poles, enc_tolerance] = unpack_cfg(motor_cfg)

    flags = uint8(motor_cfg.has_quadrature_encoder); 
    flags = bitor(flags, bitshift(uint8(motor_cfg.has_hall_sens), 1));
    resolution = motor_cfg.rotor_encoder_resolution;
    rotor_offset = motor_cfg.rotor_index_offset;
    n_poles = motor_cfg.pole_pairs * 2;
    enc_tolerance = motor_cfg.encoder_tolerance;

end
